simulink model "power_turbine"  (R2024a)
settings: Solver=ode3  StartTime=0.0  StopTime=2  FixedStep=0.0001  RelTol=1e-4
libraries: spsThreePhaseParallelRLCLoadLib x1, spsExcitationSystemLib x1, spsHydraulicTurbineandGovernorLib x1, eePowerMeasurement x1, spsSynchronousMachinepuStandardLib x1, spsThreePhaseVIMeasurementLib x1, spspowerguiLib x1
Description:
  | Copyright 2008-2009 The MathWorks(TM), Inc.
settings Model: Creator=patrice  LastModifiedBy=Aswin
settings SolverCC: AlgebraicLoopSolver=TrustRegion
settings DataIOCC: SaveFormat=Array  SignalLoggingSaveFormat=ModelDataLogs  ReturnWorkspaceOutputs=off  SignalLoggingName=sigsOut
settings OptimizationCC: BlockReduction=off  BooleanDataType=off  ExpressionDepthLimit=2147483647  InitFltsAndDblsToZero=on  EfficientMapNaN2IntZero=off  LifeSpan=inf
settings DebuggingCC: UnderspecifiedInitializationDetection=Classic  MergeDetectMultiDrivingBlocksExec=none  CheckExecutionContextPreStartOutputMsg=on  SignalResolutionControl=TryResolveAllWithWarning  MultiTaskDSMMsg=warning  MultiTaskCondExecSysMsg=none  SigSpecEnsureSampleTimeMsg=none  FcnCallInpInsideContextMsg=warning  UnconnectedInputMsg=warning  UnconnectedOutputMsg=warning  UnconnectedLineMsg=warning  StateNameClashWarn=warning  SFUnexpectedBacktrackingDiag=warning  SFNoUnconditionalDefaultTransitionDiag=warning  SFExecutionAtInitializationDiag=none  ArithmeticOperatorsInVariantConditions=warning
settings HardwareCC: ProdBitPerPointer=32  ProdBitPerSizeT=32  ProdBitPerPtrDiffT=32  ProdLargestAtomicFloat=None  ProdIntDivRoundTo=Undefined  ProdEndianess=Unspecified  ProdWordSize=32  ProdHWDeviceType=32-bit Generic  TargetUnknown=on
settings ModelReferenceCC: PropagateSignalLabelsOutOfModel=off
settings SFSimCC: SimUseLocalCustomCode=off  CustomCodeUndefinedFunction=UseInterfaceOnly
settings RTWCC: RTWUseLocalCustomCode=off  GPUComputeCapability=3.5
settings CodeAppCC: StateflowObjectComments=on
settings GRTTargetCC: TargetLangStandard=C89/C90 (ANSI)  CombineOutputUpdateFcns=off  GRTInterface=on
settings ConfigComp: CovMetricSettings=dw  CovSaveCumulativeToWorkspaceVar=on  CovSaveSingleToWorkspaceVar=on  CovExternalEMLEnable=off

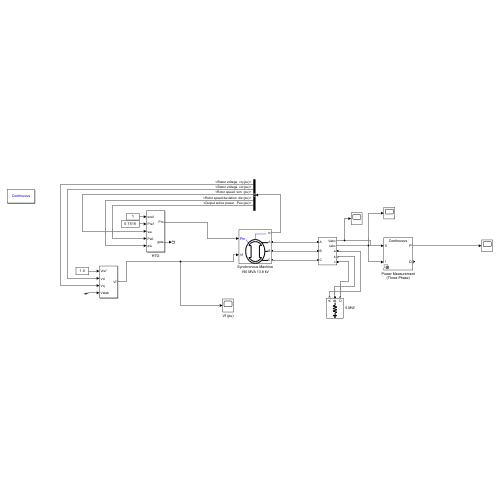
[thumbnail: Simulink's stored preview of the top-level diagram]
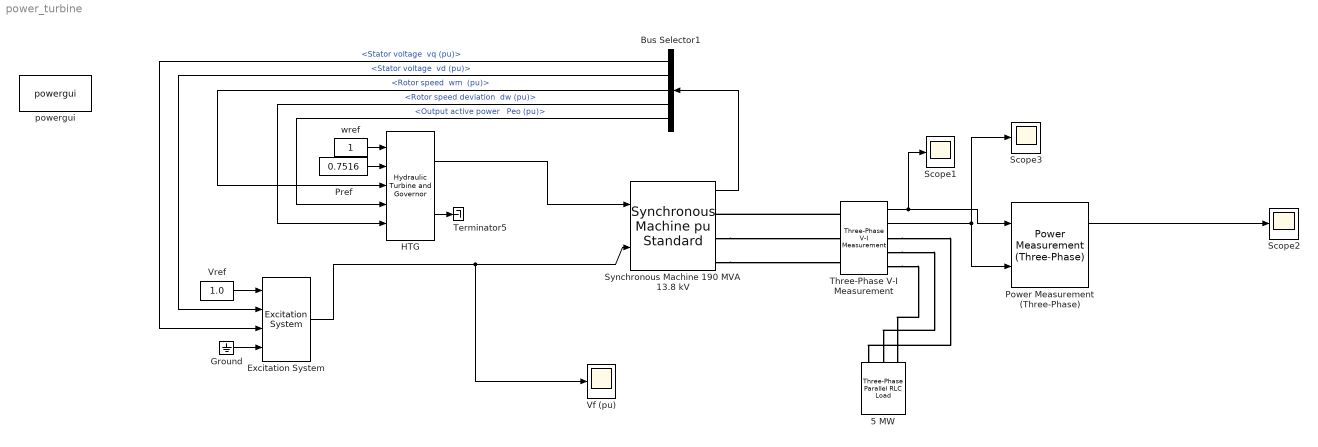
== system power_turbine ==
  5 MW : spsThreePhaseParallelRLCLoadLib/Three-Phase Parallel RLC Load  LConnTagsString=A|B|C  Configuration=Y (grounded)  NominalVoltage=7.50e3  Vabc=[1e3 1e3 1e3]  Vabcp=[1e3 1e3 1e3]  NominalFrequency=50  UnbalancedPower=off  ActivePower=5e6  InductivePower=0  CapacitivePower=0  Pabc=[10e3 9e3 11e3]  QLabc=[100 90 110]  QCabc=[100 90 110]  Pabcp=[10e3 9e3 11e3]  QLabcp=[100 90 110]  QCabcp=[100 90 110]  Measurements=Branch voltages and currents  LoadType=constant Z
  Bus Selector1 : BusSelector  OutputSignals="dq0 components.Stator voltage  vq (pu),dq0 components.Stator voltage  vd (pu),Mechanical.Rotor speed  wm  (pu),Mechanical.Rotor speed deviation  dw (pu),Output active power   Peo (pu)"
  Excitation System : spsExcitationSystemLib/Excitation System  tr=20e-3  reg=[ 300, 0.001 ]  exc=[ 1, 0 ]  tgr=[ 0, 0 ]  damp=[ 0.01, 0.1 ]  sat=[ 0, 0 ]  lim=[ -11.5, 11.5, 0 ]  v0=[1,1.2901]
      settings: LibrarySourceBlock=sps_lib/Electrical Machines/Synchronous Machine Control/Excitation System
  Ground : Ground
  HTG : spsHydraulicTurbineandGovernorLib/Hydraulic Turbine and Governor  sm="[ 10/3  0.07 ]"  gate="[  0.01  0.97518  -0.1  0.1 ]"  reg="[  0.05  1  0.2  0.1 0.01  ]"  hyd="[  0  2.67  ]"  dref=0  po=1
      settings: LibrarySourceBlock=|
      | sps_lib/Electrical Machines/Synchronous Machine Control/Hydraulic Turbine
      | and Governor
  Power Measurement (Three-Phase) : eePowerMeasurement/Power Measurement (Three-Phase)  LabelModeActiveChoice=Continuous  F=60  K=[0 1 2 3]  Seq=Positive  Ts=0
  Pref : Constant  Value=0.7516
  Scope1 : Scope
  Scope2 : Scope
  Scope3 : Scope
  Synchronous Machine 190 MVA 13.8 kV : spsSynchronousMachinepuStandardLib/Synchronous Machine pu Standard  PresetModel=No  MechanicalLoad=Mechanical power Pm  ShowDetailedParameters=on  RotorType=Salient-pole  Units=per unit standard parameters  MeasurementBus=off  NominalParameters="[ 190E6  13800   50 ]"  Reactances1=[ 31 32 33 34 35 36 37 ]  Reactances2=[ 1.305, 0.296, 0.252, 0.474, 0.243, 0.18 ]  dAxisTimeConstants=Short-circuit  qAxisTimeConstants=Open-circuit  TimeConstants1=[]  TimeConstants2=[]  TimeConstants3=[]  TimeConstants4=[]  TimeConstants5=[ 1.01, 0.053, 0.1 ]  TimeConstants6=[]  TimeConstants7=[]  TimeConstants8=[]  StatorResistance=2.8544e-3  Mechanical="[ 3.2 0  32]"  PolePairs=32  InitialConditions=[0 0 0 0 0 0 0 0 1]  SetSaturation=off  Saturation=[0.6404,0.7127,0.8441,0.9214,0.9956,1.082,1.19,1.316,1.457;0.7,0.7698,0.8872,0.9466,0.9969,1.046,1.1,1.151,1.201]  LoadFlowParameters=[1 150000000 0 0]  TsPowergui=0  TsBlock=-1  IterativeModel=Forward Euler  IterativeDiscreteModel=Trapezoidal non iterative  BusType=PV  Pref=170000000  Qref=0  Qmin=-inf  Qmax=inf  PLF=0  QLF=0
  Terminator5 : Terminator
  Three-Phase V-I Measurement : spsThreePhaseVIMeasurementLib/Three-Phase V-I Measurement  VoltageMeasurement=phase-to-ground  SetLabelV=off  LabelV=Vabc  Vpu=off  VpuLL=off  CurrentMeasurement=yes  SetLabelI=off  LabelI=Iabc  Ipu=off  Pbase=100e6  Vbase=500e3  OutputType=Complex  PhasorSimulation=off  PSBequivalent=0
  Vf (pu) : Scope
  Vref : Constant  Value=1.0
  powergui : spspowerguiLib/powergui  Priority=2  SimulationMode=Continuous  SampleTime=0  frequency=60  Iterations=50  frequencyindice=50  Pbase=100e6  ErrMax=1e-4  UnitsV=kV  UnitsW=MW  buscounter=0  FunctionMessages=off  echomessages=off  EnableUseOfTLC=off  CurrentSourceSwitches=off  DisableSnubberDevices=off  DisableRonSwitches=off  DisableVfSwitches=off  DisplayEquations=off  AutomaticDiscreteSolvers=off  SolverType=Tustin/Backward Euler (TBE)  Interpol=off  ExternalGateDelay=off  methode=off  Ts=0  x0status=blocks  SPID=off  SwTol=0  HookPort=off  NonlinearTolerance=1e-4  nMaxIteration=100  ContinueOnMaxIteration=off  RestoreLinks=warning  ResistiveCurrentMeasurement=off  Frange=logspace(0,3,50)  Ylog=off  Xlog=off  ShowGrid=off  save=off  variable=ZData  structure=0  ZoomFFT=on  StartTime=0.0  cycles=2  DisplayStyle=off  fundamental=60  FreqAxis=off  MaxFrequency=1000  frequencyindicesteady=1  RmsSteady=1  display=off
  wref : Constant
  wires:
  HTG/1 -> Synchronous Machine 190 MVA 13.8 kV/1
  Bus Selector1/2 -> Excitation System/2  "<Stator voltage  vd (pu)>"
  Ground/1 -> Excitation System/4
  Synchronous Machine 190 MVA 13.8 kV/1 -> Bus Selector1/1
  Bus Selector1/3 -> HTG/3  "<Rotor speed  wm  (pu)>"
  wref/1 -> HTG/1
  Excitation System/1 -> Synchronous Machine 190 MVA 13.8 kV/2, Vf (pu)/1
  Vref/1 -> Excitation System/1
  Pref/1 -> HTG/2
  Bus Selector1/4 -> HTG/5  "<Rotor speed deviation  dw (pu)>"
  Bus Selector1/1 -> Excitation System/3  "<Stator voltage  vq (pu)>"
  HTG/2 -> Terminator5/1
  Bus Selector1/5 -> HTG/4  "<Output active power   Peo (pu)>"
  Three-Phase V-I Measurement/1 -> Scope1/1, Power Measurement (Three-Phase)/1
  Three-Phase V-I Measurement/2 -> Power Measurement (Three-Phase)/2, Scope3/1
  Power Measurement (Three-Phase)/1 -> Scope2/1
  connections:
  Three-Phase V-I Measurement/LConn1 -- Synchronous Machine 190 MVA 13.8 kV/RConn1
  Three-Phase V-I Measurement/RConn2 -- 5 MW/LConn2
  Three-Phase V-I Measurement/RConn3 -- 5 MW/LConn3
  Synchronous Machine 190 MVA 13.8 kV/RConn3 -- Three-Phase V-I Measurement/LConn3
  Synchronous Machine 190 MVA 13.8 kV/RConn2 -- Three-Phase V-I Measurement/LConn2
  Three-Phase V-I Measurement/RConn1 -- 5 MW/LConn1
